simulink model "afe_dqctrl_inv_psm"  (R2026a)
settings: Solver=ode23t  StopTime=simlength  FixedStep=tc  MaxStep=glb_time.tc  RelTol=1e-4
values from neighbouring files (symbols this model uses):
  afe_ctrl = ctrl_afe_setup(glb_time.ts_afe, grid_emu.omega_grid_nom)    [init_model.m]
  afe_pwm_phase_shift_mod1 = 0    [init_model.m]
  CTRPIFF_CLIP_RELEASE = 0.001    [init_model.m]
  filters = setup_global_filters(glb_time.ts_afe, glb_time.ts_inv, glb_time.ts_dab, glb_time.tc)    [init_model.m]
  glb_time = timing_setup(fpwm_afe, trgo_afe, fpwm_inv, trgo_inv, fpwm_single_phase_inv, trgo_single_phase_inv, fpwm_dab, trgo_dab,      fpwm_psfbc, trgo_psfbc, fpwm_isop_rail, trgo_isop_rail, fpwm_cllc, trgo_cllc, t_measure, tc_factor, tc_decimation, delay_pwm, dead_time_afe,      dead_time_inv, dead_time_single_phase_inv, dead_time_dab, dead_time_psfbc, dead_time_isop_rail, dead_time_cllc)    [init_model.m]
  grid_emu = grid_three_phase_emulator('Dyn11', delta_star, grid_nominal_power, application_voltage, us1, us2, fgrid,                  eq_grid_inductance, eq_grid_resistance, eta, ucc, i1m, p_iron, n1, n2, core_area, core_length, mur,                  up_xi_pu_ref, up_eta_pu_ref, un_xi_pu_ref, un_eta_pu_ref)    [init_model.m]
  heatsink = liquid_cooled_plate_2kw_setup(weight, no_weight, cp_al, heat_capacity_hs, thermal_conductivity_al,      Rth_switch_HA, Rth_mosfet_HA, Rth_diode_HA, Tambient, DThs_init)    [init_model.m]
  inv_pwm_phase_shift_mod1 = 0    [init_model.m]
  ki_align = 18    [init_model.m]
  kp_align = 0.25    [init_model.m]
  lim_down_align = -0.05    [init_model.m]
  lim_up_align = 0.05    [init_model.m]
  omega_m_sim = psm.omega_m_bez    [init_model.m]
  psm = psm_calculus()    [init_model.m]
  psm_ctrl = ctrl_pmsm_setup(glb_time.ts_inv, psm.omega_bez, u_psm_scale, psm.Jm_norm)    [init_model.m]
  simlength = 1.75    [init_model.m]
  Tambient = 40    [init_model.m]
  time_gain_afe_module_1 = 1.0002    [init_model.m]
  time_gain_inv_module_2 = 1.001    [init_model.m]
  time_start_motor_control = 0.25    [init_model.m]
  torque_overload_factor = 1.15    [init_model.m]
  u_cm_comp_mod1 = 0    [init_model.m]
  u_psm_scale_ekf = sqrt(3)/2 * 2/3 * hwdata.inv.udc_nom/psm.ubez    [init_model.m]
undefined symbols (not defined in the file or in its folder): hwdata, igbt, magnitude, omega_m_bez, rpm_base, torque_base
libraries: fl_lib x99, nesl_utility x96, igbt_simple_lib x12, single_phase_transformer_lib x3, threephase_inductor_lib x2, dclink_for_two_levels x2, three_phase_pwm_modulator x2, cstblocks_lti x2, discrete_time_low_pass_filter x1, lithium_ion_battery x1, three_phase_voltage_with_frt_emulator x1, simple_flexible_shaft x1
(part 8 of 9)

== system afe_dqctrl_inv_psm/afe_dq_mod1/AFE_control/afe_control/grid_voltage_phase_lock_loops/FHT-PLL_simulink/pll_stageB/double_integrator_observer ==
  theta : Inport
  Gain : Gain  Gain=afe_ctrl.di_obs.Ldso  Multiplication=Matrix(K*u)
  Gain1 : Gain  Gain=afe_ctrl.di_obs.Adso  Multiplication=Matrix(K*u)
  Gain2 : Gain  Gain=afe_ctrl.di_obs.Cso  Multiplication=Matrix(K*u)
  Selector : Selector  InputPortWidth=2  IndexOptions=Index vector (dialog)  Indices=2  OutputSizes=1
  Sum : Sum  Inputs=-+|
  Sum1 : Sum  Inputs=|++
  Unit Delay : UnitDelay  SampleTime=-1
  bounder1 : MATLAB Function  TreatAsAtomicUnit=on
  bounder2 : MATLAB Function  TreatAsAtomicUnit=on
  omega_hat : Outport
  wires:
  bounder2/1(y) -> Sum/1  "theta_hat_bounded"
  bounder1/1(y) -> Gain/1
  theta/1 -> Sum/2  "theta"
  Unit Delay/1 -> Gain2/1, Selector/1, Gain1/1
  Sum/1 -> bounder1/1(u)  "e"
  Sum1/1 -> Unit Delay/1
  Gain1/1 -> Sum1/2
  Gain2/1 -> bounder2/1(u)  "theta_hat"
  Selector/1 -> omega_hat/1
  Gain/1 -> Sum1/1

== system afe_dqctrl_inv_psm/afe_dq_mod1/AFE_control/afe_control/grid_voltage_phase_lock_loops/dq_pll/pll_stageA/mormalization_and_transformation ==
  ug_a : Inport
  ug_b : Inport  Port=2
  ug_c : Inport  Port=3
  abc2alphabeta : MATLAB Function  TreatAsAtomicUnit=on
  ug_alpha : Outport  VectorParamsAs1DForOutWhenUnconnected=off
  ug_beta : Outport  Port=2  VectorParamsAs1DForOutWhenUnconnected=off
  wires:
  abc2alphabeta/2(beta) -> ug_beta/1  "u_grid_beta"
  abc2alphabeta/1(alpha) -> ug_alpha/1  "u_grid_alpha"
  ug_a/1 -> abc2alphabeta/1(a)
  ug_b/1 -> abc2alphabeta/2(b)
  ug_c/1 -> abc2alphabeta/3(c)

== system afe_dqctrl_inv_psm/afe_dq_mod1/AFE_control/afe_control/grid_voltage_phase_lock_loops/dq_pll/pll_stageA/sequences ==
  u_grid_alpha : Inport
  u_grid_beta : Inport  Port=2
  gamma_grid : Inport  Port=3
  Terminator : Terminator
  Terminator1 : Terminator
  alphabeta2xieta : Subsystem
  u_grid_pos_xi : Outport
  u_grid_pos_eta : Outport  Port=2
  wires:
  alphabeta2xieta/1(xi) -> u_grid_pos_xi/1  "u_grid_pos_xi"
  alphabeta2xieta/2(eta) -> u_grid_pos_eta/1  "u_grid_pos_eta"
  u_grid_alpha/1 -> alphabeta2xieta/1(alpha)  "u_grid_alpha"
  u_grid_beta/1 -> alphabeta2xieta/2(beta)  "u_grid_beta"
  gamma_grid/1 -> alphabeta2xieta/3(gamma)  "phase_grid"
  alphabeta2xieta/3(Out3) -> Terminator/1  "neg_xi"
  alphabeta2xieta/4(Out4) -> Terminator1/1  "neg_eta"

== system afe_dqctrl_inv_psm/afe_dq_mod1/AFE_control/afe_control/grid_voltage_phase_lock_loops/dq_pll/pll_stageB/double_integrator_observer ==
  phase : Inport
  Gain : Gain  Gain=afe_ctrl.di_obs.Ldso  Multiplication=Matrix(K*u)
  Gain1 : Gain  Gain=afe_ctrl.di_obs.Adso  Multiplication=Matrix(K*u)
  Gain2 : Gain  Gain=afe_ctrl.di_obs.Cso  Multiplication=Matrix(K*u)
  Selector : Selector  InputPortWidth=2  IndexOptions=Index vector (dialog)  Indices=2  OutputSizes=1
  Sum : Sum  Inputs=-+|
  Sum1 : Sum  Inputs=|++
  Unit Delay : UnitDelay  SampleTime=-1
  bounder1 : MATLAB Function  TreatAsAtomicUnit=on
  bounder2 : MATLAB Function  TreatAsAtomicUnit=on
  omega_hat : Outport
  wires:
  Gain/1 -> Sum1/1
  Selector/1 -> omega_hat/1
  Gain2/1 -> bounder2/1(u)  "theta_hat"
  Gain1/1 -> Sum1/2
  Sum1/1 -> Unit Delay/1
  Sum/1 -> bounder1/1(u)  "e"
  Unit Delay/1 -> Gain1/1, Selector/1, Gain2/1
  phase/1 -> Sum/2  "phase"
  bounder1/1(y) -> Gain/1  "e_bounded"
  bounder2/1(y) -> Sum/1  "theta_hat_bounded"

== system afe_dqctrl_inv_psm/afe_dq_mod1/AFE_control/afe_control/grid_voltage_phase_lock_loops/dq_pll/pll_stageB/scheduled-p-gain ==
  In1 : Inport
  Switch : Switch  Criteria=u2 > Threshold  Threshold=0.5  SaturateOnIntegerOverflow=off  InputSameDT=off
  kp1 : Gain  Gain=afe_ctrl.pll_p  SaturateOnIntegerOverflow=on  OutDataTypeStr=Inherit: Same as input  ParamDataTypeStr=Inherit: Same as input
  kp3 : Gain  Gain=afe_ctrl.pll_p_frt  SaturateOnIntegerOverflow=on  OutDataTypeStr=Inherit: Same as input  ParamDataTypeStr=Inherit: Same as input
  Out2 : Outport
  wires:
  kp3/1 -> Switch/1
  kp1/1 -> Switch/3
  [frt_active] -> Switch/2
  In1/1 -> kp1/1, kp3/1
  Switch/1 -> Out2/1

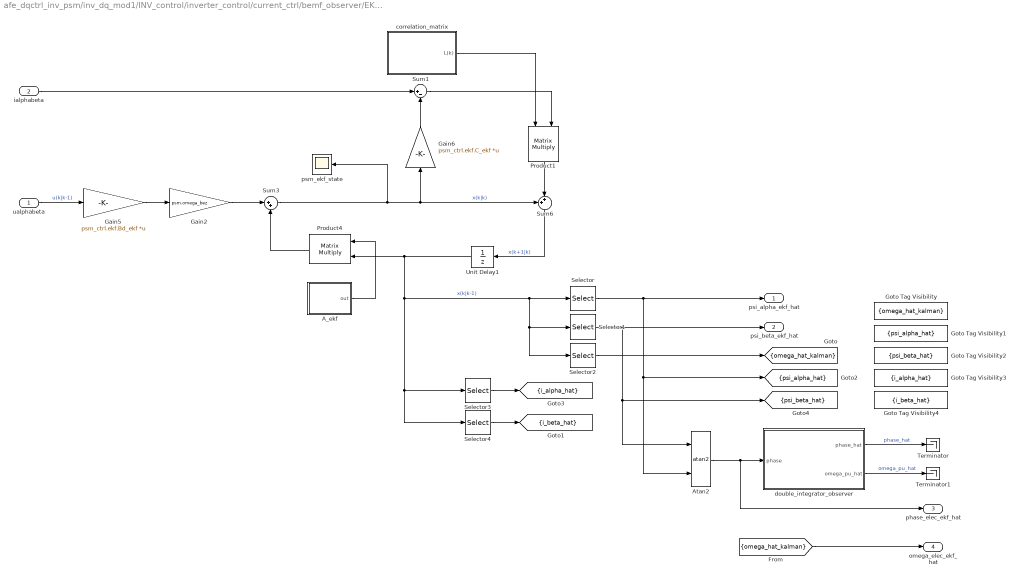
== system afe_dqctrl_inv_psm/inv_dq_mod1/INV_control/inverter_control/current_ctrl/bemf_observer/EKF_bemf_observer/extended_kalman_observer ==
  ualphabeta : Inport
  ialphabeta : Inport  Port=2
  A_ekf : Subsystem
  Atan2 : Trigonometry  Operator=atan2
  Gain2 : Gain  Gain=psm.omega_bez
  Gain5 : Gain  Gain=psm_ctrl.ekf.Bd_ekf  Multiplication=Matrix(K*u)
  Gain6 : Gain  Gain=psm_ctrl.ekf.C_ekf  Multiplication=Matrix(K*u)
  Goto Tag Visibility : GotoTagVisibility  GotoTag=omega_hat_kalman
  Goto Tag Visibility1 : GotoTagVisibility  GotoTag=psi_alpha_hat
  Goto Tag Visibility2 : GotoTagVisibility  GotoTag=psi_beta_hat
  Goto Tag Visibility3 : GotoTagVisibility  GotoTag=i_alpha_hat
  Goto Tag Visibility4 : GotoTagVisibility  GotoTag=i_beta_hat
  Product1 : Product  Multiplication=Matrix(*)
  Product4 : Product  Multiplication=Matrix(*)
  Selector : Selector  InputPortWidth=6  IndexOptions=Index vector (dialog)  Indices=3  OutputSizes=1
  Selector1 : Selector  InputPortWidth=6  IndexOptions=Index vector (dialog)  Indices=4  OutputSizes=1
  Selector2 : Selector  InputPortWidth=6  IndexOptions=Index vector (dialog)  Indices=5  OutputSizes=1
  Selector3 : Selector  InputPortWidth=6  IndexOptions=Index vector (dialog)  Indices=1  OutputSizes=1
  Selector4 : Selector  InputPortWidth=6  IndexOptions=Index vector (dialog)  Indices=2  OutputSizes=1
  Sum1 : Sum  Inputs=|+-
  Sum3 : Sum  Inputs=|++
  Sum6 : Sum  Inputs=++|
  Terminator : Terminator
  Terminator1 : Terminator
  Unit Delay1 : UnitDelay  InitialCondition=[0 0 1 1 0 0]*glb_time.ts_inv  SampleTime=-1
  correlation_matrix : Subsystem
  double_integrator_observer : Subsystem
  psm_ekf_state : Scope
      settings: ActiveDisplayYMinimum=-2.6651275002473325  ActiveDisplayYMaximum=3.9005956712949552
  psi_alpha_ekf_hat : Outport
  psi_beta_ekf_hat : Outport  Port=2
  phase_elec_ekf_hat : Outport  Port=3
  omega_elec_ekf_hat : Outport  Port=4
  tag scope: i_alpha_hat=scoped, i_beta_hat=scoped, omega_hat_kalman=scoped, psi_alpha_hat=scoped, psi_beta_hat=scoped
  wires:
  Gain5/1 -> Gain2/1
  Gain6/1 -> Sum1/2
  Sum6/1 -> Unit Delay1/1  "x(k+1|k)"
  Sum1/1 -> Product1/2
  ialphabeta/1 -> Sum1/1
  ualphabeta/1 -> Gain5/1  "u(k|k-1)"
  Sum3/1 -> psm_ekf_state/1, Gain6/1, Sum6/1  "x(k|k)"
  Unit Delay1/1 -> Selector2/1, Selector1/1, Selector/1, Selector3/1, Selector4/1, Product4/2  "x(k|k-1)"
  A_ekf/1(out) -> Product4/1
  Selector1/1 -> Atan2/1, [psi_beta_hat], psi_beta_ekf_hat/1
  Selector/1 -> Atan2/2, [psi_alpha_hat], psi_alpha_ekf_hat/1
  Selector2/1 -> [omega_hat_kalman]
  Selector3/1 -> [i_alpha_hat]
  Selector4/1 -> [i_beta_hat]
  Product4/1 -> Sum3/2
  Atan2/1 -> phase_elec_ekf_hat/1, double_integrator_observer/1(phase)
  Gain2/1 -> Sum3/1
  Product1/1 -> Sum6/2
  correlation_matrix/1(L(k)) -> Product1/1
  double_integrator_observer/1(phase_hat) -> Terminator/1  "phase_hat"
  double_integrator_observer/2(omega_pu_hat) -> Terminator1/1  "omega_pu_hat"
  [omega_hat_kalman] -> omega_elec_ekf_hat/1

== system afe_dqctrl_inv_psm/inv_dq_mod1/INV_control/inverter_control/current_ctrl/bemf_observer/bemf_observer/double_integrator_observer ==
  theta : Inport
  Dead Zone : DeadZone  LowerValue=-0.01  UpperValue=0.01
  Gain : Gain  Gain=psm_ctrl.di_obs.komega
  Gain1 : Gain  Gain=psm_ctrl.di_obs.ktheta
  Gain2 : Gain  Gain=psm.omega_bez
  Gain3 : Gain  Gain=1/psm.omega_bez
  Gain4 : Gain  Gain=glb_time.ts_inv
  Gain5 : Gain  Gain=glb_time.ts_inv
  Gain6 : Gain  Gain=glb_time.ts_inv
  Sum : Sum  Inputs=-+|
  Sum1 : Sum  Inputs=|++
  Sum2 : Sum  Inputs=|++
  Sum8 : Sum  Inputs=++|
  Unit Delay1 : UnitDelay  InitialCondition=pi  SampleTime=-1
  Unit Delay2 : UnitDelay  SampleTime=-1
  bounder1 : MATLAB Function  TreatAsAtomicUnit=on
  bounder2 : MATLAB Function  TreatAsAtomicUnit=on
  omega_pu_hat : Outport  VectorParamsAs1DForOutWhenUnconnected=off
  theta_hat : Outport  Port=2  VectorParamsAs1DForOutWhenUnconnected=off
  wires:
  Gain1/1 -> Gain6/1
  theta/1 -> Sum/2  "theta_bemf"
  Sum8/1 -> Unit Delay1/1
  Unit Delay1/1 -> bounder2/1(u)
  Sum1/1 -> Unit Delay2/1
  Gain/1 -> Gain4/1
  Unit Delay2/1 -> omega_pu_hat/1, Sum1/2, Gain5/1
  Sum2/1 -> Sum8/2
  bounder2/1(y) -> Sum2/2, theta_hat/1, Sum/1  "theta_hat"
  bounder1/1(y) -> Gain1/1, Gain/1
  Gain2/1 -> Sum8/1
  Gain3/1 -> Sum1/1
  Gain5/1 -> Gain2/1
  Sum/1 -> bounder1/1(u)
  Gain4/1 -> Gain3/1
  Gain6/1 -> Sum2/1

== system afe_dqctrl_inv_psm/inv_dq_mod1/INV_control/inverter_control/current_ctrl/bemf_observer/bemf_observer/psi_alpha_hat ==
  ualpha : Inport
  ialpha : Inport  Port=2
  udc : Inport  Port=3
  Gain1 : Gain  Gain=psm.Rs_norm
  Gain2 : Gain  Gain=psm_ctrl.emf_fb_p
  Gain3 : Gain  Gain=psm_ctrl.emf_p
  Gain4 : Gain  Gain=psm.omega_bez
  Gain5 : Gain  Gain=psm.Ls_norm
  Gain6 : Gain  Gain=psm_ctrl.u_psm_scale
  Gain7 : Gain  Gain=glb_time.ts_inv
  Product : Product  RndMeth=Zero
  Sum : Sum  Inputs=|+-
  Sum1 : Sum  Inputs=|+-
  Sum2 : Sum  Inputs=++-  SaturateOnIntegerOverflow=on
  Sum3 : Sum  Inputs=|++
  Sum4 : Sum  Inputs=+-  SaturateOnIntegerOverflow=on
  Unit Delay1 : UnitDelay  SampleTime=-1
  Unit Delay2 : UnitDelay  SampleTime=-1
  Unit Delay3 : UnitDelay  SampleTime=-1
  psi_s_alpha_hat : Outport  VectorParamsAs1DForOutWhenUnconnected=off
  psi_r_alpha_hat : Outport  Port=2  VectorParamsAs1DForOutWhenUnconnected=off
  wires:
  [psi_r_m_alpha_mod1] -> Sum1/1
  [psi_r_alpha_hat_mod1] -> Sum1/2
  Gain4/1 -> Gain7/1
  Sum2/1 -> Gain4/1
  Gain3/1 -> Sum2/3
  ialpha/1 -> Gain5/1, Gain1/1
  Gain1/1 -> Sum/2
  Sum/1 -> Sum2/2
  ualpha/1 -> Product/1
  Gain5/1 -> Unit Delay3/1
  Unit Delay1/1 -> Sum4/1, psi_s_alpha_hat/1, Gain3/1, Sum3/2
  Sum3/1 -> Unit Delay1/1
  Sum4/1 -> Unit Delay2/1
  Sum1/1 -> Gain2/1
  Gain2/1 -> Sum2/1
  Gain7/1 -> Sum3/1
  Product/1 -> Gain6/1
  Gain6/1 -> Sum/1
  Unit Delay2/1 -> psi_r_alpha_hat/1
  Unit Delay3/1 -> Sum4/2
  udc/1 -> Product/2

== system afe_dqctrl_inv_psm/inv_dq_mod1/INV_control/inverter_control/current_ctrl/bemf_observer/bemf_observer/psi_beta_hat ==
  ubeta : Inport
  ibeta : Inport  Port=2
  udc : Inport  Port=3
  Gain1 : Gain  Gain=psm.Rs_norm
  Gain2 : Gain  Gain=psm_ctrl.emf_fb_p
  Gain3 : Gain  Gain=psm_ctrl.emf_p
  Gain4 : Gain  Gain=psm.omega_bez
  Gain5 : Gain  Gain=psm.Ls_norm
  Gain6 : Gain  Gain=psm_ctrl.u_psm_scale
  Gain7 : Gain  Gain=glb_time.ts_inv
  Product : Product  RndMeth=Zero
  Sum : Sum  Inputs=|+-
  Sum1 : Sum  Inputs=|+-
  Sum2 : Sum  Inputs=++-  SaturateOnIntegerOverflow=on
  Sum3 : Sum  Inputs=|++
  Sum4 : Sum  Inputs=+-  SaturateOnIntegerOverflow=on
  Unit Delay1 : UnitDelay  SampleTime=-1
  Unit Delay2 : UnitDelay  SampleTime=-1
  Unit Delay3 : UnitDelay  SampleTime=-1
  psi_s_beta_hat : Outport  VectorParamsAs1DForOutWhenUnconnected=off
  psi_r_beta_hat : Outport  Port=2  VectorParamsAs1DForOutWhenUnconnected=off
  wires:
  Gain5/1 -> Unit Delay3/1
  Sum/1 -> Sum2/2
  Gain1/1 -> Sum/2
  ibeta/1 -> Gain5/1, Gain1/1
  Gain3/1 -> Sum2/3
  Sum2/1 -> Gain4/1
  Gain4/1 -> Gain7/1
  Sum1/1 -> Gain2/1
  [psi_r_beta_hat_mod1] -> Sum1/2
  [psi_r_m_beta_mod1] -> Sum1/1
  Unit Delay1/1 -> Gain3/1, Sum4/1, psi_s_beta_hat/1, Sum3/2
  Sum3/1 -> Unit Delay1/1
  Sum4/1 -> Unit Delay2/1
  Gain2/1 -> Sum2/1
  ubeta/1 -> Product/1
  Gain7/1 -> Sum3/1
  Product/1 -> Gain6/1
  Gain6/1 -> Sum/1
  Unit Delay2/1 -> psi_r_beta_hat/1
  Unit Delay3/1 -> Sum4/2
  udc/1 -> Product/2

== system afe_dqctrl_inv_psm/inv_dq_mod1/INV_control/inverter_control/current_ctrl/bemf_observer/bemf_observer/theta_bemf_hat ==
  psi_r_alpha_hat : Inport
  psi_r_beta_hat : Inport  Port=2
  Trigonometric Function : Trigonometry  Operator=atan2  OutputSignalType=real
  theta_emf_hat : Outport  VectorParamsAs1DForOutWhenUnconnected=off
  wires:
  psi_r_alpha_hat/1 -> Trigonometric Function/2
  psi_r_beta_hat/1 -> Trigonometric Function/1
  Trigonometric Function/1 -> theta_emf_hat/1

== system afe_dqctrl_inv_psm/inv_dq_mod1/INV_control/inverter_control/current_ctrl/bemf_observer/bemf_observer_ccaller/Reset Trigger ==
  Step : Step  Time=0.01  InitialValue=1  FinalValue=0
  Out1 : Outport
  wires:
  Step/1 -> Out1/1  "Reset"

== system afe_dqctrl_inv_psm/inv_dq_mod1/INV_control/inverter_control/current_ctrl/current_ctrl/dq_pi_with_vector_antiwindup mod1/dq_vector_pi ==
  id : Inport
  id_ref : Inport  Port=2
  iq : Inport  Port=3
  iq_ref : Inport  Port=4
  Sum1 : Sum  Inputs=|-+
  Sum2 : Sum  Inputs=|-+
  bounder1 : Subsystem
  bounder2 : Subsystem
  pi_d : Subsystem
  pi_q : Subsystem
  switch : Subsystem
  vector lenght : Subsystem
  md_sat : Outport
  mq_sat : Outport  Port=2
  wires:
  bounder2/2(clip) -> switch/2(clip 2)
  vector lenght/2(m) -> bounder1/3(m), bounder2/1(m)
  Sum2/1 -> pi_q/1(iq_tilde)
  pi_d/1(ud_out) -> vector lenght/1(md), bounder1/1(md)
  pi_q/1(Vqs_out) -> bounder2/3(mq), vector lenght/2(mq)
  vector lenght/1(m_1) -> bounder1/2(m_1), bounder2/2(m_1)
  switch/1(clip) -> pi_q/2(clip), pi_d/2(clip)
  iq/1 -> Sum2/1
  Sum1/1 -> pi_d/1(id_tilde)
  bounder1/2(clip) -> switch/1(clip 1)
  id/1 -> Sum1/1
  bounder1/1(md_sat) -> md_sat/1
  bounder2/1(mq_sat) -> mq_sat/1
  id_ref/1 -> Sum1/2
  iq_ref/1 -> Sum2/2

== system afe_dqctrl_inv_psm/inv_dq_mod1/INV_control/inverter_control/current_ctrl/current_ctrl/dq_pi_with_vector_antiwindup mod1/dq_vector_pi_ccaller ==
  id : Inport
  id_ref : Inport  Port=2
  iq : Inport  Port=3
  iq_ref : Inport  Port=4
  udc_pu : Inport  Port=5
  Bus Selector : BusSelector  OutputSignals=ud,uq
  C Caller : CCaller  FunctionName=dqvector_pi_process_simulink  PortSpecificationStruct="%)30     .    ,!8   8    (     @         %    \"     T    !     0         %  0 \"0    $    _    07)G3F%M90  4&]R=$YA;64 4V-O<&4     26YD97@     5'EP90      4VEZ90      27-';&]B86P   X    P    !@    @    $          4    (     0    ,    !         !   P!O=70 #@   #     &    \"     0         !0    @    !     P    $         $  # &]U=  .    .     8    (    !          %    \"     $    &     0         0   ...(+7280 chars)"
  Constant : Constant  Value=glb_time.ts_inv
  Constant1 : Constant  Value=psm_ctrl.kp_i
  Constant2 : Constant  Value=psm_ctrl.ki_i
  Constant3 : Constant
  Constant4 : Constant  Value=psm_ctrl.kp_i
  Constant5 : Constant  Value=psm_ctrl.ki_i
  Data Type Conversion{,1..2,4..6,9..13} (11 alike) : DataTypeConversion  OutDataTypeStr=single  SaturateOnIntegerOverflow=off  RndMeth=Floor
  Data Type Conversion3 : DataTypeConversion  OutDataTypeStr=double  SaturateOnIntegerOverflow=off  RndMeth=Floor
  Data Type Conversion7 : DataTypeConversion  OutDataTypeStr=double  SaturateOnIntegerOverflow=off  RndMeth=Floor
  Data Type Conversion8 : DataTypeConversion  OutDataTypeStr=uint8  SaturateOnIntegerOverflow=off  RndMeth=Floor
  Reset : Subsystem
  ud_ctrl_out : Outport
  uq_ctrl_out : Outport  Port=2
  wires:
  Data Type Conversion5/1 -> C Caller/6
  Data Type Conversion/1 -> C Caller/2
  C Caller/1 -> Bus Selector/1  "out"
  Data Type Conversion1/1 -> C Caller/3
  Data Type Conversion4/1 -> C Caller/5
  Data Type Conversion2/1 -> C Caller/4
  Data Type Conversion6/1 -> C Caller/7
  Bus Selector/2 -> Data Type Conversion3/1  "<uq>"
  Bus Selector/1 -> Data Type Conversion7/1  "<ud>"
  Data Type Conversion7/1 -> ud_ctrl_out/1  "ud"
  Data Type Conversion3/1 -> uq_ctrl_out/1  "uq"
  Data Type Conversion8/1 -> C Caller/1
  Data Type Conversion9/1 -> C Caller/8
  Data Type Conversion10/1 -> C Caller/9
  Data Type Conversion11/1 -> C Caller/12
  Data Type Conversion13/1 -> C Caller/10
  Data Type Conversion12/1 -> C Caller/11
  Constant3/1 -> Data Type Conversion11/1
  Constant5/1 -> Data Type Conversion12/1
  Constant4/1 -> Data Type Conversion13/1
  Constant2/1 -> Data Type Conversion10/1
  Constant1/1 -> Data Type Conversion9/1
  Constant/1 -> Data Type Conversion6/1
  udc_pu/1 -> Data Type Conversion5/1
  iq/1 -> Data Type Conversion4/1
  iq_ref/1 -> Data Type Conversion2/1
  Reset/1(en) -> Data Type Conversion8/1
  id_ref/1 -> Data Type Conversion/1
  id/1 -> Data Type Conversion1/1

== system afe_dqctrl_inv_psm/inv_dq_mod1/inverter/inverter/three_phase_inverter_with_igbt_simple/three_phase_inverter_with_igbt_simple/igbt_simple_1/IGBT_simple ==
  IGBT_SIMPLE Simplified IGBT + antiparallel FWD : igbt_simple_lib/IGBT_SIMPLE Simplified IGBT + antiparallel FWD  Vce_sat=vce_sat_m V  Vf=v_gamma_m V  Vth=Vth_gate_m V  Vhyst=Vth_gate_hyst_m V  Ron=rce_on_m mOhm  Rd=rd_on_m mOhm  Goff=Gce_off_m 1/Ohm  i_specify=off  i_priority=None  i=0 A  i_nominal_specify=off  i_nominal_value=1  i_nominal_unit=A  v_specify=off  v_priority=None  v=0 V  v_nominal_specify=off  v_nominal_value=1  v_nominal_unit=V  i_t_specify=off  i_t_priority=None  i_t=0 A  i_t_nominal_specify=off  i_t_nominal_value=1  i_t_nominal_unit=A  i_d_specify=off  i_d_priority=None  i_d=0 A  i_d_nominal_specify=off  i_d_nominal_value=1  i_d_nominal_unit=A
  iph1 : nesl_utility/PS-Simulink Converter  PhysicalDomain=network_engine_domain  SubClassName=ps_output  LeftPortType=input  RightPortType=output  PseudoPeriodic=off  Frequencies=[]  VectorFormat=1-D array  Unit=A  AffineConversion=off
  iph2 : nesl_utility/PS-Simulink Converter  PhysicalDomain=network_engine_domain  SubClassName=ps_output  LeftPortType=input  RightPortType=output  PseudoPeriodic=off  Frequencies=[]  VectorFormat=1-D array  Unit=A  AffineConversion=off
  G : PMIOPort  Side=Left
  C : PMIOPort  Port=2  Side=Left
  E : PMIOPort  Port=3  Side=Right
  tag scope: diode_current_Q1=scoped, igbt_current_Q1=scoped
  wires:
  iph1/1 -> [igbt_current_Q1]  "i_device_thermal_inv"
  iph2/1 -> [diode_current_Q1]  "i_device_thermal_inv"
  connections:
  IGBT_SIMPLE Simplified IGBT + antiparallel FWD/RConn1 -- E/RConn1
  IGBT_SIMPLE Simplified IGBT + antiparallel FWD/LConn1 -- C/RConn1
  IGBT_SIMPLE Simplified IGBT + antiparallel FWD/LConn2 -- G/RConn1
  IGBT_SIMPLE Simplified IGBT + antiparallel FWD/RConn2 -- iph1/LConn1
  IGBT_SIMPLE Simplified IGBT + antiparallel FWD/RConn3 -- iph2/LConn1

== system afe_dqctrl_inv_psm/inv_dq_mod1/inverter/inverter/three_phase_inverter_with_igbt_simple/three_phase_inverter_with_igbt_simple/igbt_simple_2/IGBT_simple ==
  IGBT_SIMPLE Simplified IGBT + antiparallel FWD : igbt_simple_lib/IGBT_SIMPLE Simplified IGBT + antiparallel FWD  Vce_sat=vce_sat_m V  Vf=v_gamma_m V  Vth=Vth_gate_m V  Vhyst=Vth_gate_hyst_m V  Ron=rce_on_m mOhm  Rd=rd_on_m mOhm  Goff=Gce_off_m 1/Ohm  i_specify=off  i_priority=None  i=0 A  i_nominal_specify=off  i_nominal_value=1  i_nominal_unit=A  v_specify=off  v_priority=None  v=0 V  v_nominal_specify=off  v_nominal_value=1  v_nominal_unit=V  i_t_specify=off  i_t_priority=None  i_t=0 A  i_t_nominal_specify=off  i_t_nominal_value=1  i_t_nominal_unit=A  i_d_specify=off  i_d_priority=None  i_d=0 A  i_d_nominal_specify=off  i_d_nominal_value=1  i_d_nominal_unit=A
  iph1 : nesl_utility/PS-Simulink Converter  PhysicalDomain=network_engine_domain  SubClassName=ps_output  LeftPortType=input  RightPortType=output  PseudoPeriodic=off  Frequencies=[]  VectorFormat=1-D array  Unit=A  AffineConversion=off
  iph2 : nesl_utility/PS-Simulink Converter  PhysicalDomain=network_engine_domain  SubClassName=ps_output  LeftPortType=input  RightPortType=output  PseudoPeriodic=off  Frequencies=[]  VectorFormat=1-D array  Unit=A  AffineConversion=off
  G : PMIOPort  Side=Left
  C : PMIOPort  Port=2  Side=Left
  E : PMIOPort  Port=3  Side=Right
  tag scope: diode_current_Q2=scoped, igbt_current_Q2=scoped
  wires:
  iph1/1 -> [igbt_current_Q2]  "i_device_thermal_inv"
  iph2/1 -> [diode_current_Q2]  "i_device_thermal_inv"
  connections:
  IGBT_SIMPLE Simplified IGBT + antiparallel FWD/RConn1 -- E/RConn1
  IGBT_SIMPLE Simplified IGBT + antiparallel FWD/LConn1 -- C/RConn1
  IGBT_SIMPLE Simplified IGBT + antiparallel FWD/LConn2 -- G/RConn1
  IGBT_SIMPLE Simplified IGBT + antiparallel FWD/RConn2 -- iph1/LConn1
  IGBT_SIMPLE Simplified IGBT + antiparallel FWD/RConn3 -- iph2/LConn1

== system afe_dqctrl_inv_psm/inv_dq_mod1/inverter/inverter/three_phase_inverter_with_igbt_simple/three_phase_inverter_with_igbt_simple/igbt_simple_3/IGBT_simple ==
  IGBT_SIMPLE Simplified IGBT + antiparallel FWD : igbt_simple_lib/IGBT_SIMPLE Simplified IGBT + antiparallel FWD  Vce_sat=vce_sat_m V  Vf=v_gamma_m V  Vth=Vth_gate_m V  Vhyst=Vth_gate_hyst_m V  Ron=rce_on_m mOhm  Rd=rd_on_m mOhm  Goff=Gce_off_m 1/Ohm  i_specify=off  i_priority=None  i=0 A  i_nominal_specify=off  i_nominal_value=1  i_nominal_unit=A  v_specify=off  v_priority=None  v=0 V  v_nominal_specify=off  v_nominal_value=1  v_nominal_unit=V  i_t_specify=off  i_t_priority=None  i_t=0 A  i_t_nominal_specify=off  i_t_nominal_value=1  i_t_nominal_unit=A  i_d_specify=off  i_d_priority=None  i_d=0 A  i_d_nominal_specify=off  i_d_nominal_value=1  i_d_nominal_unit=A
  iph1 : nesl_utility/PS-Simulink Converter  PhysicalDomain=network_engine_domain  SubClassName=ps_output  LeftPortType=input  RightPortType=output  PseudoPeriodic=off  Frequencies=[]  VectorFormat=1-D array  Unit=A  AffineConversion=off
  iph2 : nesl_utility/PS-Simulink Converter  PhysicalDomain=network_engine_domain  SubClassName=ps_output  LeftPortType=input  RightPortType=output  PseudoPeriodic=off  Frequencies=[]  VectorFormat=1-D array  Unit=A  AffineConversion=off
  G : PMIOPort  Side=Left
  C : PMIOPort  Port=2  Side=Left
  E : PMIOPort  Port=3  Side=Right
  tag scope: diode_current_Q3=scoped, igbt_current_Q3=scoped
  wires:
  iph1/1 -> [igbt_current_Q3]  "i_device_thermal_inv"
  iph2/1 -> [diode_current_Q3]  "i_device_thermal_inv"
  connections:
  IGBT_SIMPLE Simplified IGBT + antiparallel FWD/RConn1 -- E/RConn1
  IGBT_SIMPLE Simplified IGBT + antiparallel FWD/LConn1 -- C/RConn1
  IGBT_SIMPLE Simplified IGBT + antiparallel FWD/LConn2 -- G/RConn1
  IGBT_SIMPLE Simplified IGBT + antiparallel FWD/RConn2 -- iph1/LConn1
  IGBT_SIMPLE Simplified IGBT + antiparallel FWD/RConn3 -- iph2/LConn1

== system afe_dqctrl_inv_psm/inv_dq_mod1/inverter/inverter/three_phase_inverter_with_igbt_simple/three_phase_inverter_with_igbt_simple/igbt_simple_4/IGBT_simple ==
  IGBT_SIMPLE Simplified IGBT + antiparallel FWD : igbt_simple_lib/IGBT_SIMPLE Simplified IGBT + antiparallel FWD  Vce_sat=vce_sat_m V  Vf=v_gamma_m V  Vth=Vth_gate_m V  Vhyst=Vth_gate_hyst_m V  Ron=rce_on_m mOhm  Rd=rd_on_m mOhm  Goff=Gce_off_m 1/Ohm  i_specify=off  i_priority=None  i=0 A  i_nominal_specify=off  i_nominal_value=1  i_nominal_unit=A  v_specify=off  v_priority=None  v=0 V  v_nominal_specify=off  v_nominal_value=1  v_nominal_unit=V  i_t_specify=off  i_t_priority=None  i_t=0 A  i_t_nominal_specify=off  i_t_nominal_value=1  i_t_nominal_unit=A  i_d_specify=off  i_d_priority=None  i_d=0 A  i_d_nominal_specify=off  i_d_nominal_value=1  i_d_nominal_unit=A
  iph1 : nesl_utility/PS-Simulink Converter  PhysicalDomain=network_engine_domain  SubClassName=ps_output  LeftPortType=input  RightPortType=output  PseudoPeriodic=off  Frequencies=[]  VectorFormat=1-D array  Unit=A  AffineConversion=off
  iph2 : nesl_utility/PS-Simulink Converter  PhysicalDomain=network_engine_domain  SubClassName=ps_output  LeftPortType=input  RightPortType=output  PseudoPeriodic=off  Frequencies=[]  VectorFormat=1-D array  Unit=A  AffineConversion=off
  G : PMIOPort  Side=Left
  C : PMIOPort  Port=2  Side=Left
  E : PMIOPort  Port=3  Side=Right
  tag scope: diode_current_Q4=scoped, igbt_current_Q4=scoped
  wires:
  iph1/1 -> [igbt_current_Q4]  "i_device_thermal_inv"
  iph2/1 -> [diode_current_Q4]  "i_device_thermal_inv"
  connections:
  IGBT_SIMPLE Simplified IGBT + antiparallel FWD/RConn1 -- E/RConn1
  IGBT_SIMPLE Simplified IGBT + antiparallel FWD/LConn1 -- C/RConn1
  IGBT_SIMPLE Simplified IGBT + antiparallel FWD/LConn2 -- G/RConn1
  IGBT_SIMPLE Simplified IGBT + antiparallel FWD/RConn2 -- iph1/LConn1
  IGBT_SIMPLE Simplified IGBT + antiparallel FWD/RConn3 -- iph2/LConn1

== system afe_dqctrl_inv_psm/inv_dq_mod1/inverter/inverter/three_phase_inverter_with_igbt_simple/three_phase_inverter_with_igbt_simple/igbt_simple_5/IGBT_simple ==
  IGBT_SIMPLE Simplified IGBT + antiparallel FWD : igbt_simple_lib/IGBT_SIMPLE Simplified IGBT + antiparallel FWD  Vce_sat=vce_sat_m V  Vf=v_gamma_m V  Vth=Vth_gate_m V  Vhyst=Vth_gate_hyst_m V  Ron=rce_on_m mOhm  Rd=rd_on_m mOhm  Goff=Gce_off_m 1/Ohm  i_specify=off  i_priority=None  i=0 A  i_nominal_specify=off  i_nominal_value=1  i_nominal_unit=A  v_specify=off  v_priority=None  v=0 V  v_nominal_specify=off  v_nominal_value=1  v_nominal_unit=V  i_t_specify=off  i_t_priority=None  i_t=0 A  i_t_nominal_specify=off  i_t_nominal_value=1  i_t_nominal_unit=A  i_d_specify=off  i_d_priority=None  i_d=0 A  i_d_nominal_specify=off  i_d_nominal_value=1  i_d_nominal_unit=A
  iph1 : nesl_utility/PS-Simulink Converter  PhysicalDomain=network_engine_domain  SubClassName=ps_output  LeftPortType=input  RightPortType=output  PseudoPeriodic=off  Frequencies=[]  VectorFormat=1-D array  Unit=A  AffineConversion=off
  iph2 : nesl_utility/PS-Simulink Converter  PhysicalDomain=network_engine_domain  SubClassName=ps_output  LeftPortType=input  RightPortType=output  PseudoPeriodic=off  Frequencies=[]  VectorFormat=1-D array  Unit=A  AffineConversion=off
  G : PMIOPort  Side=Left
  C : PMIOPort  Port=2  Side=Left
  E : PMIOPort  Port=3  Side=Right
  tag scope: diode_current_Q5=scoped, igbt_current_Q5=scoped
  wires:
  iph1/1 -> [igbt_current_Q5]  "i_device_thermal_inv"
  iph2/1 -> [diode_current_Q5]  "i_device_thermal_inv"
  connections:
  IGBT_SIMPLE Simplified IGBT + antiparallel FWD/RConn1 -- E/RConn1
  IGBT_SIMPLE Simplified IGBT + antiparallel FWD/LConn1 -- C/RConn1
  IGBT_SIMPLE Simplified IGBT + antiparallel FWD/LConn2 -- G/RConn1
  IGBT_SIMPLE Simplified IGBT + antiparallel FWD/RConn2 -- iph1/LConn1
  IGBT_SIMPLE Simplified IGBT + antiparallel FWD/RConn3 -- iph2/LConn1

== system afe_dqctrl_inv_psm/inv_dq_mod1/inverter/inverter/three_phase_inverter_with_igbt_simple/three_phase_inverter_with_igbt_simple/igbt_simple_6/IGBT_simple ==
  IGBT_SIMPLE Simplified IGBT + antiparallel FWD : igbt_simple_lib/IGBT_SIMPLE Simplified IGBT + antiparallel FWD  Vce_sat=vce_sat_m V  Vf=v_gamma_m V  Vth=Vth_gate_m V  Vhyst=Vth_gate_hyst_m V  Ron=rce_on_m mOhm  Rd=rd_on_m mOhm  Goff=Gce_off_m 1/Ohm  i_specify=off  i_priority=None  i=0 A  i_nominal_specify=off  i_nominal_value=1  i_nominal_unit=A  v_specify=off  v_priority=None  v=0 V  v_nominal_specify=off  v_nominal_value=1  v_nominal_unit=V  i_t_specify=off  i_t_priority=None  i_t=0 A  i_t_nominal_specify=off  i_t_nominal_value=1  i_t_nominal_unit=A  i_d_specify=off  i_d_priority=None  i_d=0 A  i_d_nominal_specify=off  i_d_nominal_value=1  i_d_nominal_unit=A
  iph1 : nesl_utility/PS-Simulink Converter  PhysicalDomain=network_engine_domain  SubClassName=ps_output  LeftPortType=input  RightPortType=output  PseudoPeriodic=off  Frequencies=[]  VectorFormat=1-D array  Unit=A  AffineConversion=off
  iph2 : nesl_utility/PS-Simulink Converter  PhysicalDomain=network_engine_domain  SubClassName=ps_output  LeftPortType=input  RightPortType=output  PseudoPeriodic=off  Frequencies=[]  VectorFormat=1-D array  Unit=A  AffineConversion=off
  G : PMIOPort  Side=Left
  C : PMIOPort  Port=2  Side=Left
  E : PMIOPort  Port=3  Side=Right
  tag scope: diode_current_Q6=scoped, igbt_current_Q6=scoped
  wires:
  iph1/1 -> [igbt_current_Q6]  "i_device_thermal_inv"
  iph2/1 -> [diode_current_Q6]  "i_device_thermal_inv"
  connections:
  IGBT_SIMPLE Simplified IGBT + antiparallel FWD/RConn1 -- E/RConn1
  IGBT_SIMPLE Simplified IGBT + antiparallel FWD/LConn1 -- C/RConn1
  IGBT_SIMPLE Simplified IGBT + antiparallel FWD/LConn2 -- G/RConn1
  IGBT_SIMPLE Simplified IGBT + antiparallel FWD/RConn2 -- iph1/LConn1
  IGBT_SIMPLE Simplified IGBT + antiparallel FWD/RConn3 -- iph2/LConn1

== system afe_dqctrl_inv_psm/afe_dq_mod1/AFE_control/afe_control/grid_voltage_phase_lock_loops/FHT-PLL/pll_stageA/filter_and_transformation/FHTalpha ==
  u : Inport
  Bus Selector : BusSelector  OutputSignals=output_pu_hat,output_pu_hat_dot
  C Caller : CCaller  FunctionName=first_harmonic_tracker_process_simulink  PortSpecificationStruct="%)30     .    B \\   8    (     @         %    \"     D    !     0         %  0 \"0    $    _    07)G3F%M90  4&]R=$YA;64 4V-O<&4     26YD97@     5'EP90      4VEZ90      27-';&]B86P   X    P    !@    @    $          4    (     0    ,    !         !   P!O=70 #@   #     &    \"     0         !0    @    !     P    $         $  # &]U=  .    .     8    (    !          %    \"     $    &     0         0  ...(+4988 chars)"
  Constant : Constant  Value=glb_time.ts_afe
  Constant1 : Constant  Value=12
  Constant4 : Constant  Value=afe_ctrl.fht_grid.omega_fht
  Constant5 : Constant  Value=afe_ctrl.fht_grid.delta_fht
  Constant6 : Constant  Value=afe_ctrl.fht_grid.Ld_fht(1)
  Constant7 : Constant  Value=afe_ctrl.fht_grid.Ld_fht(2)
  Data Type Conversion{1..2,6..9} (6 alike) : DataTypeConversion  OutDataTypeStr=single  SaturateOnIntegerOverflow=off  RndMeth=Floor
  Data Type Conversion10 : DataTypeConversion  OutDataTypeStr=double  SaturateOnIntegerOverflow=off  RndMeth=Floor
  Data Type Conversion3 : DataTypeConversion  OutDataTypeStr=uint8  SaturateOnIntegerOverflow=off  RndMeth=Floor
  Data Type Conversion4 : DataTypeConversion  OutDataTypeStr=double  SaturateOnIntegerOverflow=off  RndMeth=Floor
  Data Type Conversion5 : DataTypeConversion  OutDataTypeStr=uint8  SaturateOnIntegerOverflow=off  RndMeth=Floor
  Gain : Gain  Gain=1/afe_ctrl.fht_grid.omega_fht
  Step : Step  Time=0.0125  InitialValue=1  FinalValue=0
  ud_hat : Outport
  uq_hat : Outport  Port=2
  wires:
  Data Type Conversion9/1 -> C Caller/7
  Data Type Conversion8/1 -> C Caller/6
  Data Type Conversion7/1 -> C Caller/5
  Data Type Conversion6/1 -> C Caller/4
  Data Type Conversion5/1 -> C Caller/8
  Constant5/1 -> Data Type Conversion7/1
  Constant7/1 -> Data Type Conversion9/1
  Constant6/1 -> Data Type Conversion8/1
  Constant4/1 -> Data Type Conversion6/1
  Constant1/1 -> Data Type Conversion5/1
  Constant/1 -> Data Type Conversion1/1
  u/1 -> Data Type Conversion2/1
  Step/1 -> Data Type Conversion3/1
  Bus Selector/1 -> Data Type Conversion4/1  "<output_pu_hat>"
  C Caller/1 -> Bus Selector/1
  Data Type Conversion2/1 -> C Caller/2
  Data Type Conversion1/1 -> C Caller/3
  Data Type Conversion3/1 -> C Caller/1
  Data Type Conversion4/1 -> ud_hat/1
  Data Type Conversion10/1 -> Gain/1
  Bus Selector/2 -> Data Type Conversion10/1  "<output_pu_hat_dot>"
  Gain/1 -> uq_hat/1
